simulink model "sf_debouncer_STT"  (R2025b)
settings: Solver=FixedStepDiscrete  StartTime=0.0  StopTime=10.0  RelTol=1e-3  EnableMultiTasking=on
libraries: simulink x1
settings Model: Creator=The MathWorks, Inc.  LastModifiedBy=The MathWorks, Inc.
settings SolverCC: AlgebraicLoopSolver=TrustRegion
settings DataIOCC: LimitDataPoints=on  SaveFormat=Array  ReturnWorkspaceOutputs=off
settings OptimizationCC: ReuseModelBlockBuffer=off  ExpressionDepthLimit=2147483647.0  LifeSpan=1  EfficientTunableParamExpr=on
settings DebuggingCC: ReadBeforeWriteMsg=DisableAll  WriteAfterWriteMsg=DisableAll  WriteAfterReadMsg=DisableAll  UnderspecifiedInitializationDetection=Classic  MergeDetectMultiDrivingBlocksExec=none  SolverPrmCheckMsg=warning  UnconnectedInputMsg=warning  UnconnectedOutputMsg=warning  UnconnectedLineMsg=warning  AllowSymbolicDim=off  StateNameClashWarn=warning  SFUnexpectedBacktrackingDiag=warning  SFNoUnconditionalDefaultTransitionDiag=warning  SFExecutionAtInitializationDiag=none  ArithmeticOperatorsInVariantConditions=warning
settings HardwareCC: ProdBitPerPointer=32.0  ProdBitPerSizeT=32.0  ProdBitPerPtrDiffT=32.0  ProdLargestAtomicFloat=None  ProdIntDivRoundTo=Undefined  ProdEndianess=Unspecified  ProdWordSize=32.0  ProdHWDeviceType=32-bit Generic
settings ModelReferenceCC: EnableRefExpFcnMdlSchedulingChecks=on  PropagateSignalLabelsOutOfModel=off
settings SFSimCC: SimUseLocalCustomCode=off  CustomCodeUndefinedFunction=UseInterfaceOnly
settings RTWCC: SystemTargetFile=ert.tlc  TemplateMakefile=ert_default_tmf  RTWUseLocalCustomCode=off  GPUComputeCapability=3.5  Description=Embedded Coder
settings CodeAppCC: IgnoreCustomStorageClasses=off  CustomSymbolStrModelFcn=$N  StateflowObjectComments=on
settings ERTTargetCC: InlinedParameterPlacement=Hierarchical  ERTCustomFileTemplate=example_file_process.tlc  ConvertIfToSwitch=off  SuppressUnreachableDefaultCases=off  DynamicArrayContainerType=coder::array  MultiwordLength=2048.0  GenerateSampleERTMain=on
settings ConfigComp: CovMetricSettings=dw  CovSaveCumulativeToWorkspaceVar=on  CovSaveSingleToWorkspaceVar=on  CovExternalEMLEnable=off

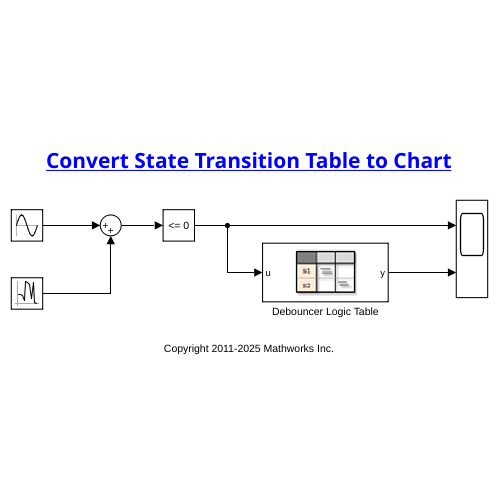
[thumbnail: Simulink's stored preview of the top-level diagram]
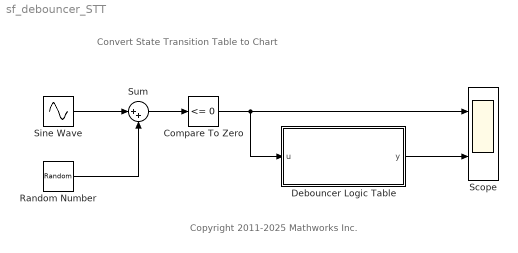
== system sf_debouncer_STT ==
  note: Copyright 2011-2025 Mathworks Inc.
  note: Convert State Transition Table to Chart
  Compare To Zero : simulink/Logic and Bit Operations/Compare To Zero  relop=<=  OutDataTypeStr=boolean
  Debouncer Logic Table : State Transition Table  TreatAsAtomicUnit=on
  Random Number : RandomNumber  Variance=0.005  SampleTime=0.01
  Scope : Scope  NumInputPorts=2
      settings: ActiveDisplayYMinimum=-5  ActiveDisplayYMaximum=5
  Sine Wave : Sin  SampleTime=0
  Sum : Sum  Inputs=|++
  wires:
  Sine Wave/1 -> Sum/1
  Random Number/1 -> Sum/2
  Sum/1 -> Compare To Zero/1
  Compare To Zero/1 -> Debouncer Logic Table/1(u), Scope/1
  Debouncer Logic Table/1(y) -> Scope/2

== stateflow chart sf_debouncer_STT/Debouncer Logic Table ==
  state ON
    en: y = 1;
  state ON_TO_OFF
  state OFF_TO_ON
  state OFF
    en: y = 0;
  (default) -> ON
  (junction 30) -> ON
  (junction 32) -> (junction 30)
  ON -> ON_TO_OFF : [u == 0]
  ON_TO_OFF -> ON [order 2] : [u == 1]
  ON_TO_OFF -> (junction 25) [order 1] : after(0.1,sec)
  (junction 25) -> (junction 23)
  OFF_TO_ON -> (junction 32) [order 1] : after(0.1,sec)
  OFF_TO_ON -> OFF [order 2] : [u == 0]
  OFF -> OFF_TO_ON : [u == 1]
  (junction 23) -> OFF
  data: u input; y output
